simulink model "can2_mcu_status_unpack"  (R2026b)
settings: Solver=VariableStepAuto
undefined symbols (not defined in the file or in its folder): P
libraries: simulink x1, svdutilitieslib x1
settings Model: Creator=aomar  LastModifiedBy=aomar

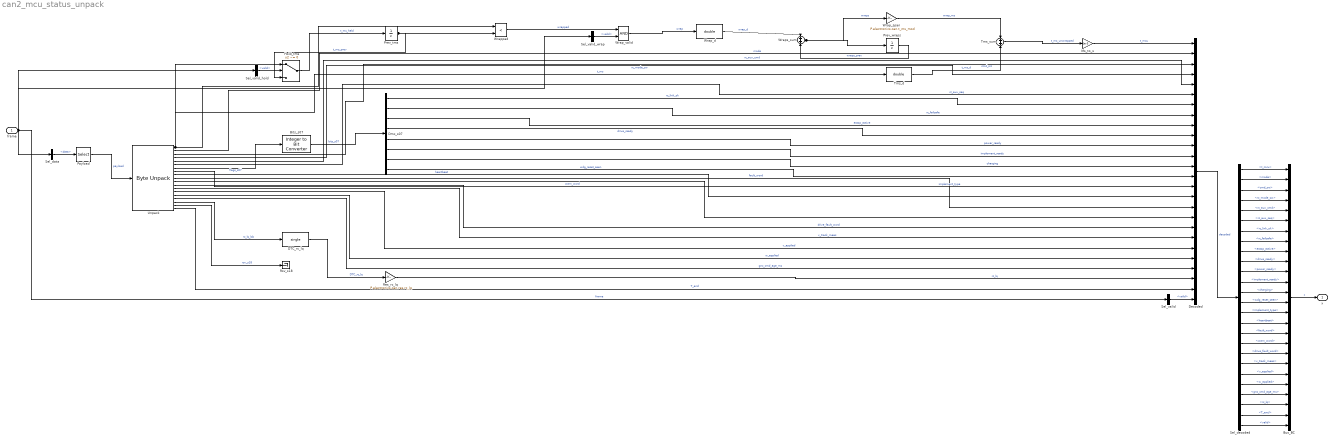
== system can2_mcu_status_unpack ==
  frame : Inport  OutDataTypeStr=Bus: Bus_CanFrame64
  Bits_s07 : simulink/Logic and Bit Operations/Integer to Bit Converter  nbits=8  signedInputValues=Unsigned  bitOrder=LSB first  outDtype=boolean
      settings: LibrarySourceBlock=|
      | commutil2/Integer to Bit
      | Converter
  Bus_BC : BusCreator  Inputs=26  OutDataTypeStr=Bus: Bus_McuStatus  NonVirtualBus=on
      settings: InheritFromInputs=off
  DTC_rc_lq : DataTypeConversion  OutDataTypeStr=single  SaturateOnIntegerOverflow=off  RndMeth=Floor
  Decoded : BusCreator  Inputs=26
  Dmx_s07 : Demux  Outputs=8
  Hold_tms : Switch  Criteria=u2 ~= 0  SaturateOnIntegerOverflow=off  InputSameDT=off
  Ms_to_s : Gain  Gain=1e-3
  Payload : Selector  InputPortWidth=64  IndexOptions=Index vector (dialog)  Indices=1:48  OutputSizes=1
  Prev_tms : UnitDelay  SampleTime=-1
  Prev_wraps : UnitDelay  SampleTime=-1
  Res_rc_lq : Gain  Gain=P.electronics.can.res.rc_lq  OutDataTypeStr=single  ParamDataTypeStr=Inherit: Same as input
  Rsv_s18 : Terminator
  Sel_data : BusSelector  OutputSignals=data
  Sel_decoded : BusSelector  OutputSignals=t_mcu,mode,cmd_src,rc_mode_sw,rc_aux_cmd,rc_aux_seq,rc_link_ok,rc_failsafe,estop_active,drive_ready,power_ready,implement_ready,charging,wdg_reset_seen,implement_type,heartbeat,fault_word,warn_word,drive_fault_word,v_track_meas,v_applied,w_applied,gnc_cmd_age_ms,rc_lq,T_encl,valid
  Sel_valid : BusSelector  OutputSignals=valid
  Sel_valid_hold : BusSelector  OutputSignals=valid
  Sel_valid_wrap : BusSelector  OutputSignals=valid
  Tms_d : DataTypeConversion  OutDataTypeStr=double  SaturateOnIntegerOverflow=off  RndMeth=Floor
  Tms_sum : Sum
  Unpack : svdutilitieslib/Byte Unpack  dimensions={1,1,1,1,1,1,1,1,1,1,1,1,2,1,1,1,1,1,1}  datatypes={'uint32','uint8','uint8','uint8','uint8','uint8','uint8','uint8','uint8','uint32','uint32','uint32','single','single','single','uint16','uint8','uint8','single'}  byteAlign=1  blockPlatform=arduinoert
      settings: LibrarySourceBlock=mcblib/Signal Management/Byte Unpack
  Wrap_d : DataTypeConversion  OutDataTypeStr=double  SaturateOnIntegerOverflow=off  RndMeth=Floor
  Wrap_span : Gain  Gain=P.electronics.can.t_ms_mod
  Wrap_valid : Logic  AllPortsSameDT=off  OutDataTypeStr=boolean
  Wrapped : RelationalOperator  Operator=<  OutDataTypeStr=boolean  RndMeth=Simplest  InputSameDT=off
  Wraps_sum : Sum
  x : Outport  OutDataTypeStr=Bus: Bus_McuStatus
  wires:
  frame/1 -> Sel_valid/1, Sel_valid_wrap/1, Sel_valid_hold/1, Sel_data/1  "frame"
  Sel_data/1 -> Payload/1  "<data>"
  Payload/1 -> Unpack/1  "payload"
  Unpack/1 -> Wrapped/1, Hold_tms/1, Tms_d/1  "t_ms"
  Unpack/2 -> Decoded/2  "mode"
  Unpack/3 -> Decoded/3  "cmd_src"
  Unpack/4 -> Decoded/4  "rc_mode_sw"
  Unpack/5 -> Decoded/5  "rc_aux_cmd"
  Unpack/6 -> Decoded/6  "rc_aux_seq"
  Unpack/7 -> Bits_s07/1  "flags_s07"
  Unpack/8 -> Decoded/15  "implement_type"
  Unpack/9 -> Decoded/16  "heartbeat"
  Unpack/10 -> Decoded/17  "fault_word"
  Unpack/11 -> Decoded/18  "warn_word"
  Unpack/12 -> Decoded/19  "drive_fault_word"
  Unpack/13 -> Decoded/20  "v_track_meas"
  Unpack/14 -> Decoded/21  "v_applied"
  Unpack/15 -> Decoded/22  "w_applied"
  Unpack/16 -> Decoded/23  "gnc_cmd_age_ms"
  Unpack/17 -> DTC_rc_lq/1  "rc_lq_lsb"
  Unpack/18 -> Rsv_s18/1  "rsv_s18"
  Unpack/19 -> Decoded/25  "T_encl"
  Sel_valid_hold/1 -> Hold_tms/2  "<valid>"
  Hold_tms/1 -> Prev_tms/1  "t_ms_held"
  DTC_rc_lq/1 -> Res_rc_lq/1  "DTC_rc_lq"
  Bits_s07/1 -> Dmx_s07/1  "bits_s07"
  Dmx_s07/1 -> Decoded/7  "rc_link_ok"
  Dmx_s07/2 -> Decoded/8  "rc_failsafe"
  Dmx_s07/3 -> Decoded/9  "estop_active"
  Dmx_s07/4 -> Decoded/10  "drive_ready"
  Dmx_s07/5 -> Decoded/11  "power_ready"
  Dmx_s07/6 -> Decoded/12  "implement_ready"
  Dmx_s07/7 -> Decoded/13  "charging"
  Dmx_s07/8 -> Decoded/14  "wdg_reset_seen"
  Res_rc_lq/1 -> Decoded/24  "rc_lq"
  Prev_tms/1 -> Hold_tms/3, Wrapped/2  "t_ms_prev"
  Wrapped/1 -> Wrap_valid/1  "wrapped"
  Sel_valid_wrap/1 -> Wrap_valid/2  "<valid>"
  Wrap_valid/1 -> Wrap_d/1  "wrap"
  Wrap_d/1 -> Wraps_sum/1  "wrap_d"
  Wraps_sum/1 -> Wrap_span/1, Prev_wraps/1  "wraps"
  Wrap_span/1 -> Tms_sum/1  "wrap_ms"
  Prev_wraps/1 -> Wraps_sum/2  "wraps_prev"
  Tms_d/1 -> Tms_sum/2  "t_ms_d"
  Tms_sum/1 -> Ms_to_s/1  "t_ms_unwrapped"
  Ms_to_s/1 -> Decoded/1  "t_mcu"
  Sel_valid/1 -> Decoded/26  "<valid>"
  Decoded/1 -> Sel_decoded/1  "decoded"
  Sel_decoded/1 -> Bus_BC/1  "<t_mcu>"
  Sel_decoded/2 -> Bus_BC/2  "<mode>"
  Sel_decoded/3 -> Bus_BC/3  "<cmd_src>"
  Sel_decoded/4 -> Bus_BC/4  "<rc_mode_sw>"
  Sel_decoded/5 -> Bus_BC/5  "<rc_aux_cmd>"
  Sel_decoded/6 -> Bus_BC/6  "<rc_aux_seq>"
  Sel_decoded/7 -> Bus_BC/7  "<rc_link_ok>"
  Sel_decoded/8 -> Bus_BC/8  "<rc_failsafe>"
  Sel_decoded/9 -> Bus_BC/9  "<estop_active>"
  Sel_decoded/10 -> Bus_BC/10  "<drive_ready>"
  Sel_decoded/11 -> Bus_BC/11  "<power_ready>"
  Sel_decoded/12 -> Bus_BC/12  "<implement_ready>"
  Sel_decoded/13 -> Bus_BC/13  "<charging>"
  Sel_decoded/14 -> Bus_BC/14  "<wdg_reset_seen>"
  Sel_decoded/15 -> Bus_BC/15  "<implement_type>"
  Sel_decoded/16 -> Bus_BC/16  "<heartbeat>"
  Sel_decoded/17 -> Bus_BC/17  "<fault_word>"
  Sel_decoded/18 -> Bus_BC/18  "<warn_word>"
  Sel_decoded/19 -> Bus_BC/19  "<drive_fault_word>"
  Sel_decoded/20 -> Bus_BC/20  "<v_track_meas>"
  Sel_decoded/21 -> Bus_BC/21  "<v_applied>"
  Sel_decoded/22 -> Bus_BC/22  "<w_applied>"
  Sel_decoded/23 -> Bus_BC/23  "<gnc_cmd_age_ms>"
  Sel_decoded/24 -> Bus_BC/24  "<rc_lq>"
  Sel_decoded/25 -> Bus_BC/25  "<T_encl>"
  Sel_decoded/26 -> Bus_BC/26  "<valid>"
  Bus_BC/1 -> x/1  "x"
